simulink model "AGC_script"  (R2024b)
settings: Solver=VariableStepAuto  StartTime=0.0  StopTime=simTim  RelTol=1e-3
libraries: dspvision x3, audiomeasurements x3
settings Model: Creator=Pedro  LastModifiedBy=Pedro

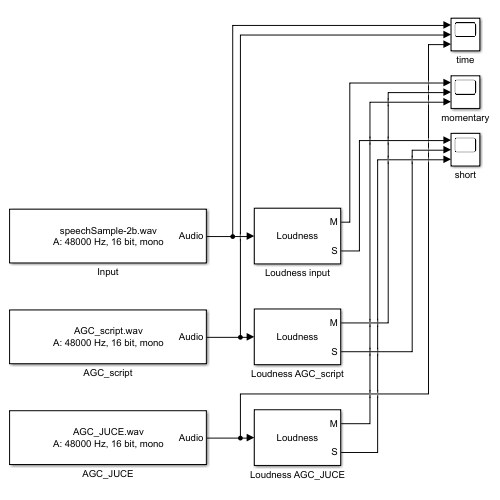
[thumbnail: Simulink's stored preview of the top-level diagram]
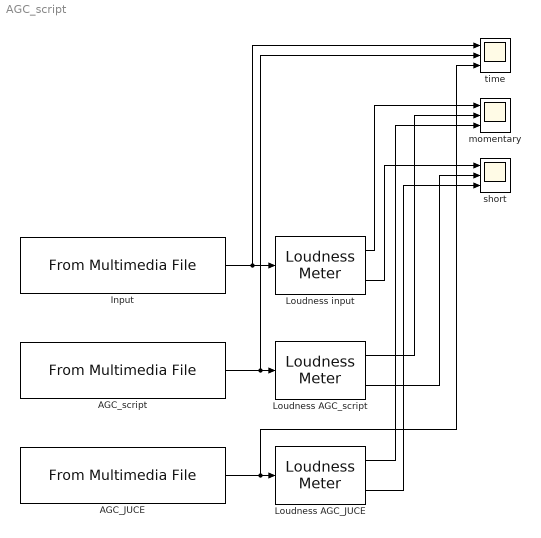
== system AGC_script ==
  AGC_JUCE : dspvision/From Multimedia File  inputFilename=C:\Users\Pedro\My Drive\25.1\Projeto Integrador\MATLAB\teste-4\AGC_JUCE.wav  readRange=[1 Inf]  loop=on  numPlays=inf  outputStreams=Audio only  videoDataType=single  audioDataType=double  inheritSampleTime=on  userDefinedSampleTime=1/30  noAudioOutput=off  isIntensityVideo=off  fourcc=RGB  colorVideoFormat=Separate color signals  outputEOF=off  dataOrg=Column-major  audioFrameSize=1024  computeAudioFrameSize=off  outSamplingMode=Sample based
      settings: LibrarySourceBlock=audiosources/From Multimedia File
  AGC_script : dspvision/From Multimedia File  inputFilename=C:\Users\Pedro\My Drive\25.1\Projeto Integrador\MATLAB\teste-4\AGC_script.wav  readRange=[1 Inf]  loop=on  numPlays=inf  outputStreams=Audio only  videoDataType=single  audioDataType=double  inheritSampleTime=on  userDefinedSampleTime=1/30  noAudioOutput=off  isIntensityVideo=off  fourcc=RGB  colorVideoFormat=Separate color signals  outputEOF=off  dataOrg=Column-major  audioFrameSize=1024  computeAudioFrameSize=off  outSamplingMode=Sample based
      settings: LibrarySourceBlock=audiosources/From Multimedia File
  Input : dspvision/From Multimedia File  inputFilename=C:\Users\Pedro\My Drive\25.1\Projeto Integrador\MATLAB\teste-4\samples\speechSample-2b.wav  readRange=[1 Inf]  loop=on  numPlays=inf  outputStreams=Audio only  videoDataType=single  audioDataType=double  inheritSampleTime=on  userDefinedSampleTime=1/30  noAudioOutput=off  isIntensityVideo=off  fourcc=RGB  colorVideoFormat=Separate color signals  outputEOF=off  dataOrg=Column-major  audioFrameSize=1024  computeAudioFrameSize=off  outSamplingMode=Sample based
      settings: LibrarySourceBlock=audiosources/From Multimedia File
  Loudness AGC_JUCE : audiomeasurements/Loudness Meter  ChannelWeights=[ 1, 1, 1, 1.41, 1.41 ]  UseRelativeScale=off  TargetLoudness=-23.0  OutputTruePeak=off  InheritSampleRate=off  SampleRate=48000  SimulateUsing=Interpreted execution
  Loudness AGC_script : audiomeasurements/Loudness Meter  ChannelWeights=[ 1, 1, 1, 1.41, 1.41 ]  UseRelativeScale=off  TargetLoudness=-23.0  OutputTruePeak=off  InheritSampleRate=off  SampleRate=48000  SimulateUsing=Interpreted execution
  Loudness input : audiomeasurements/Loudness Meter  ChannelWeights=[ 1, 1, 1, 1.41, 1.41 ]  UseRelativeScale=off  TargetLoudness=-23.0  OutputTruePeak=off  InheritSampleRate=off  SampleRate=48000  SimulateUsing=Interpreted execution
  momentary : Scope  NumInputPorts=3
  short : Scope  NumInputPorts=3
  time : Scope  NumInputPorts=3
  wires:
  AGC_JUCE/1 -> time/3, Loudness AGC_JUCE/1
  AGC_script/1 -> time/2, Loudness AGC_script/1
  Input/1 -> time/1, Loudness input/1
  Loudness AGC_JUCE/2 -> short/3
  Loudness input/1 -> momentary/1
  Loudness AGC_script/1 -> momentary/2
  Loudness AGC_JUCE/1 -> momentary/3
  Loudness input/2 -> short/1
  Loudness AGC_script/2 -> short/2
